simulink model "simLpvssDtTest"  (R2020a)
settings: Solver=FixedStepAuto  StartTime=0.0  StopTime=10  FixedStep=Ts  RelTol=1e-3
values from neighbouring files (symbols this model uses):
  P1 = lpvss(P1l)    [simulinkCoreTest.m]
  P1l = drss(nx,ny,nu);P1l.Ts = Ts    [simulinkCoreTest.m]
  P2 = lpvss(Ag,Bg,Cg,Dg,Ts)    [simulinkCoreTest.m]
  P3 = lpvlfr(Delta,G)    [simulinkCoreTest.m]
  Ts = 0.1    [simulinkCoreTest.m]
  x0 = randn(nx,1)    [simulinkCoreTest.m]
libraries: lpvcoreLibraryCore x3
settings Model: Creator=Patrick  LastModifiedBy=Patrick
settings DataIOCC: SaveOutput=off  SignalLogging=off  DSMLogging=off  SaveTime=off
settings DebuggingCC: AlgebraicLoopMsg=none

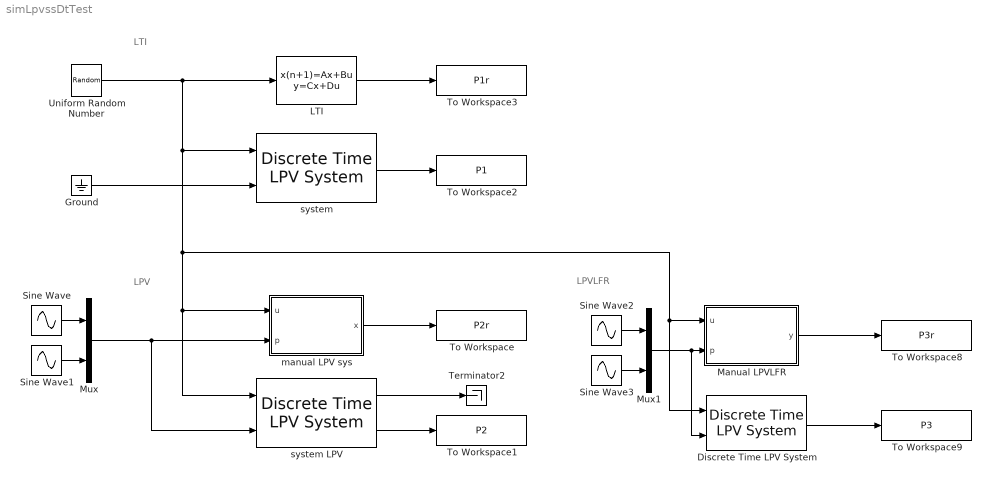
== system simLpvssDtTest ==
  note: LPV
  note: LTI
  note: LPVLFR
  Discrete Time LPV System : lpvcoreLibraryCore/Systems/Discrete Time LPV System  P=P3  x0=0  stateOut=off
      settings: SourceProductName=LPVcore
  Ground : Ground
  LTI : DiscreteStateSpace  A=P1l.A  B=P1l.B  C=P1l.C  D=P1l.D  InitialCondition=x0  SampleTime=Ts
  Manual LPVLFR : Subsystem
  Mux : Mux  Inputs=2
  Mux1 : Mux  Inputs=2
  Sine Wave : Sin  SampleTime=0
  Sine Wave1 : Sin  Frequency=2  SampleTime=0
  Sine Wave2 : Sin  Amplitude=5e-2  SampleTime=Ts
  Sine Wave3 : Sin  Amplitude=5e-2  Frequency=2  SampleTime=Ts
  Terminator2 : Terminator
  To Workspace : ToWorkspace  VariableName=P2r  SampleTime=-1
  To Workspace1 : ToWorkspace  VariableName=P2  SampleTime=-1
  To Workspace2 : ToWorkspace  VariableName=P1  SampleTime=-1
  To Workspace3 : ToWorkspace  VariableName=P1r  SampleTime=-1
  To Workspace8 : ToWorkspace  VariableName=P3r  SampleTime=-1
  To Workspace9 : ToWorkspace  VariableName=P3  SampleTime=-1
  Uniform Random Number : UniformRandomNumber  SampleTime=Ts
  manual LPV sys : Subsystem
  system : lpvcoreLibraryCore/Systems/Discrete Time LPV System  P=P1  x0=x0  stateOut=off
      settings: SourceProductName=LPVcore
  system LPV : lpvcoreLibraryCore/Systems/Discrete Time LPV System  P=P2  x0=0  stateOut=on
      settings: SourceProductName=LPVcore
  wires:
  Ground/1 -> system/2
  manual LPV sys/1(x) -> To Workspace/1
  Uniform Random Number/1 -> LTI/1, system/1, Discrete Time LPV System/1, Manual LPVLFR/1(u), system LPV/1, manual LPV sys/1(u)
  LTI/1 -> To Workspace3/1
  system/1 -> To Workspace2/1
  Sine Wave1/1 -> Mux/2
  Sine Wave/1 -> Mux/1
  Mux/1 -> system LPV/2, manual LPV sys/2(p)
  Sine Wave3/1 -> Mux1/2
  Sine Wave2/1 -> Mux1/1
  Mux1/1 -> Manual LPVLFR/2(p), Discrete Time LPV System/2
  Manual LPVLFR/1(y) -> To Workspace8/1
  Discrete Time LPV System/1 -> To Workspace9/1
  system LPV/2 -> To Workspace1/1
  system LPV/1 -> Terminator2/1

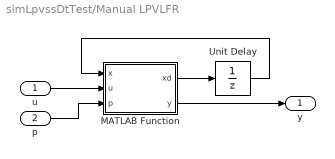
== system simLpvssDtTest/Manual LPVLFR ==
  u : Inport
  p : Inport  Port=2
  MATLAB Function : MATLAB Function  TreatAsAtomicUnit=on
  Unit Delay : UnitDelay  SampleTime=-1  HasFrameUpgradeWarning=on
  y : Outport
  wires:
  u/1 -> MATLAB Function/2(u)
  MATLAB Function/1(xd) -> Unit Delay/1
  Unit Delay/1 -> MATLAB Function/1(x)
  p/1 -> MATLAB Function/3(p)
  MATLAB Function/2(y) -> y/1

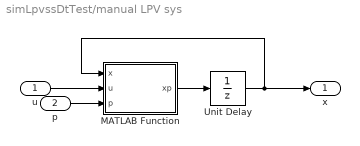
== system simLpvssDtTest/manual LPV sys ==
  u : Inport
  p : Inport  Port=2
  MATLAB Function : MATLAB Function  TreatAsAtomicUnit=on
  Unit Delay : UnitDelay  InitialCondition=[0;0]  SampleTime=Ts  HasFrameUpgradeWarning=on
  x : Outport
  wires:
  u/1 -> MATLAB Function/2(u)
  MATLAB Function/1(xp) -> Unit Delay/1
  Unit Delay/1 -> x/1, MATLAB Function/1(x)
  p/1 -> MATLAB Function/3(p)

== matlab function simLpvssDtTest/Manual LPVLFR/MATLAB Function ==
  data: x input size=2; u input; xd output size=2; p input; y output
function [xd,y] = fcn(x,u,p)
A0 = diag([.5 -.2]);
Bw = [1 3;2 6];
Bu = [1;1];
Cz = [1 3];
Cy = [2 1];
Dzw = [-1 -1];
Dzu = 3;
Dyw = [2 3];
Dyu = 5;
Delta = @(p1,p2) [p1;p2];
Deltap = Delta(p(1),p(2));
Mid = Deltap/(1-Dzw*Deltap);

A = A0+Bw*Mid*Cz;
B = Bu+Bw*Mid*Dzu;
C = Cy+Dyw*Mid*Cz;
D = Dyu+Dyw*Mid*Dzu;

xd = A*x+B*u;
y = C*x+D*u;

== matlab function simLpvssDtTest/manual LPV sys/MATLAB Function ==
  data: x input size=2; u input; xp output size=2; p input
function xp = fcn(x,u,p)
xp = zeros(2,1);
xp(1) = 0.8*x(2);
xp(2) = 0.1*p(1)*x(1)+0.5*x(2)*p(2)+u;
